simulink model "PRPM_FDM_Communication_System"  (R2024b)
settings: Solver=VariableStepAuto  StartTime=0.0  StopTime=0.2  RelTol=1e-3
libraries: commseqgen3 x4
settings Model: Creator=Aditya Narayan  LastModifiedBy=Aditya Narayan

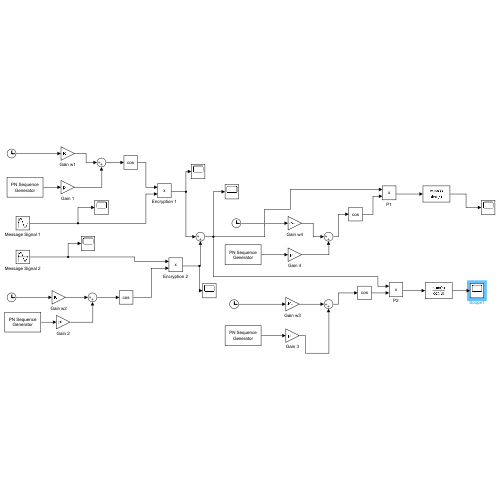
[thumbnail: Simulink's stored preview of the top-level diagram]
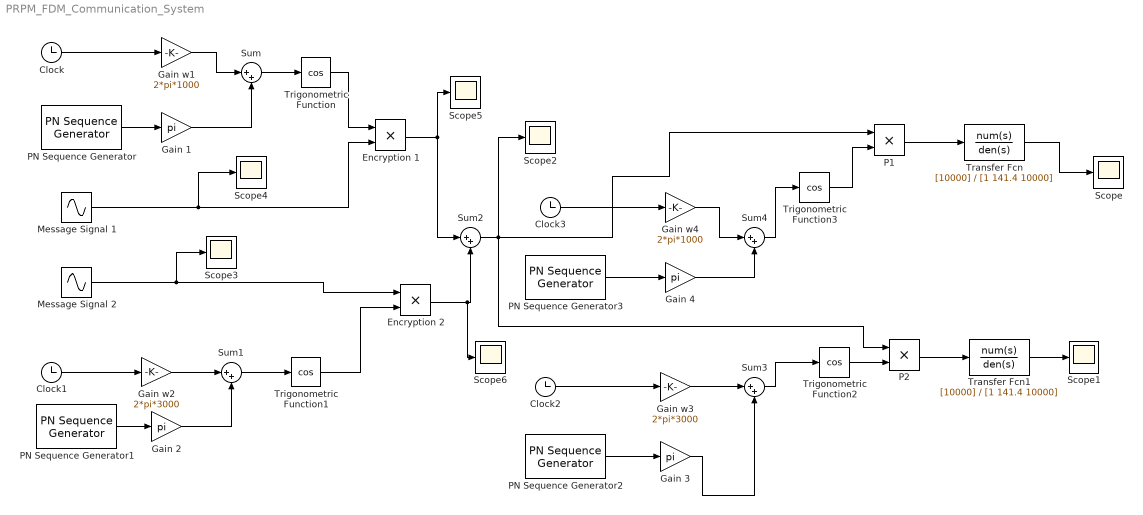
== system PRPM_FDM_Communication_System ==
  Clock{,1..3} (4 alike) : Clock
  Encryption 1 : Product
  Encryption 2 : Product
  Gain {1..4} (4 alike) : Gain  Gain=pi
  Gain w1 : Gain  Gain=2*pi*1000
  Gain w2 : Gain  Gain=2*pi*3000
  Gain w3 : Gain  Gain=2*pi*3000
  Gain w4 : Gain  Gain=2*pi*1000
  Message Signal 1 : Sin  Frequency=2*pi*50  SampleTime=0
  Message Signal 2 : Sin  Frequency=2*pi*100  SampleTime=0
  P1 : Product
  P2 : Product
  PN Sequence Generator{,1..3} (4 alike) : commseqgen3/PN Sequence Generator  poly=[5 2 0]  ini_sta=[1 0 0 0 1]  outBitMaskSource=Dialog parameter  shift=0  outVarSiz=off  maxOutSizeMode=Dialog parameter  maxOutSize=[10 1]  Ts=0.0001  sampPerFrame=1  reset=off  bitPackedOutputs=off  outDataType=double  numPackedBits=8  bitPackDataSigned=off  bitPackedOutDType=double
  Scope{,1..6} (7 alike) : Scope
  Sum{,1..4} (5 alike) : Sum  Inputs=|++
  Transfer Fcn : TransferFcn  Numerator=[10000]  Denominator=[1 141.4 10000]
  Transfer Fcn1 : TransferFcn  Numerator=[10000]  Denominator=[1 141.4 10000]
  Trigonometric Function{,1..3} (4 alike) : Trigonometry  Operator=cos
  wires:
  PN Sequence Generator/1 -> Gain 1/1
  Clock/1 -> Gain w1/1
  Gain w1/1 -> Sum/1
  Gain 1/1 -> Sum/2
  Sum/1 -> Trigonometric Function/1
  Trigonometric Function/1 -> Encryption 1/1
  Message Signal 1/1 -> Scope4/1, Encryption 1/2
  PN Sequence Generator1/1 -> Gain 2/1
  Clock1/1 -> Gain w2/1
  Gain w2/1 -> Sum1/1
  Gain 2/1 -> Sum1/2
  Sum1/1 -> Trigonometric Function1/1
  Message Signal 2/1 -> Scope3/1, Encryption 2/1
  Trigonometric Function1/1 -> Encryption 2/2
  Encryption 1/1 -> Scope5/1, Sum2/1
  Encryption 2/1 -> Scope6/1, Sum2/2
  PN Sequence Generator3/1 -> Gain 4/1
  Gain w4/1 -> Sum4/1
  Sum4/1 -> Trigonometric Function3/1
  Clock3/1 -> Gain w4/1
  Gain 4/1 -> Sum4/2
  Trigonometric Function3/1 -> P1/2
  Transfer Fcn/1 -> Scope/1
  Sum2/1 -> P2/1, Scope2/1, P1/1
  P1/1 -> Transfer Fcn/1
  Gain 3/1 -> Sum3/2
  PN Sequence Generator2/1 -> Gain 3/1
  Sum3/1 -> Trigonometric Function2/1
  Clock2/1 -> Gain w3/1
  Trigonometric Function2/1 -> P2/2
  Gain w3/1 -> Sum3/1
  P2/1 -> Transfer Fcn1/1
  Transfer Fcn1/1 -> Scope1/1
